simulink model "pmsm_mpc_simulink"  (R2022b)
settings: Solver=ode4  StartTime=0.0  StopTime=2  FixedStep=1e-05  RelTol=1e-3
values from neighbouring files (symbols this model uses):
  fault = evalin('base', 'fault')    [run_simulink_simulation.m]
  motor = evalin('base', 'motor')    [run_simulink_mpc_simulation.m]
  profile = evalin('base', 'profile')    [run_simulink_mpc_simulation.m]    (also in run_simulink_simulation.m)
settings Model: Creator=arpankailashgupta  LastModifiedBy=arpankailashgupta
settings DataIOCC: SaveOutput=off

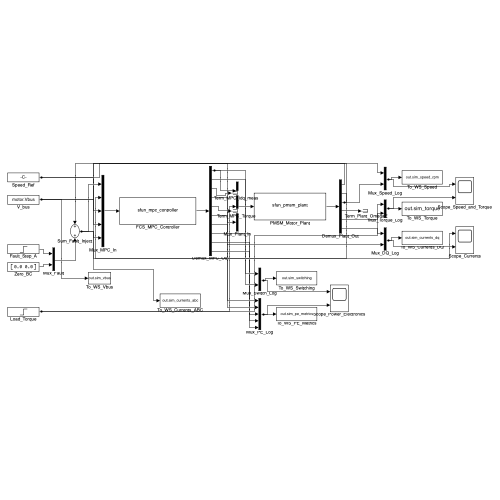
[thumbnail: Simulink's stored preview of the top-level diagram]
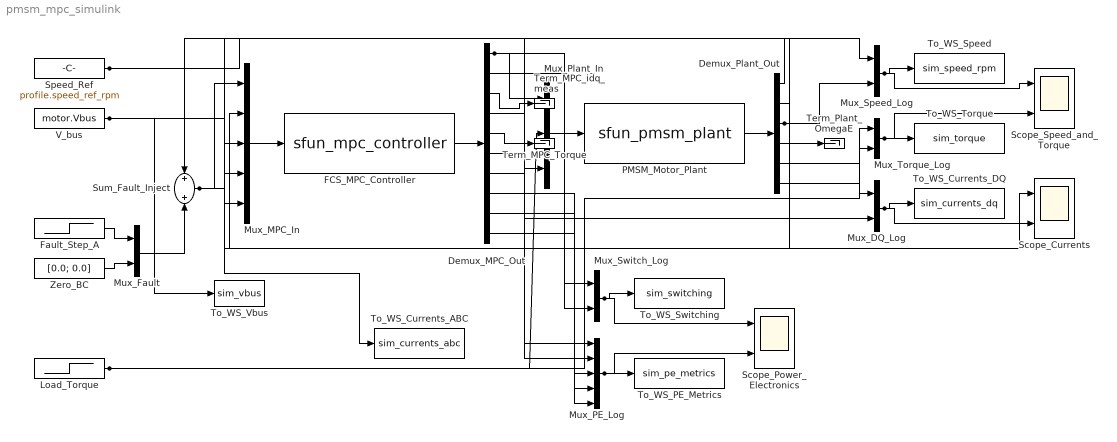
== system pmsm_mpc_simulink ==
  Demux_MPC_Out : Demux  Outputs=[3, 1, 2, 2, 1, 1, 1, 1, 1, 1]
  Demux_Plant_Out : Demux  Outputs=[3, 1, 1, 1, 1, 2]
  FCS_MPC_Controller : S-Function  FunctionName=sfun_mpc_controller  Parameters=sim_cfg.Ts_ctrl  SFunctionDeploymentMode=off  EnableBusSupport=off
  Fault_Step_A : Step  Time=fault.onset_time  Before=0.0  After=fault.offset_val * fault.enable  SampleTime=0
  Load_Torque : Step  Time=profile.load_step_time  Before=0.0  After=profile.load_torque_Nm  SampleTime=0
  Mux_DQ_Log : Mux  Inputs=2
  Mux_Fault : Mux  Inputs=2
  Mux_MPC_In : Mux  Inputs=5
  Mux_PE_Log : Mux  Inputs=5
  Mux_Plant_In : Mux  Inputs=3
  Mux_Speed_Log : Mux  Inputs=2
  Mux_Switch_Log : Mux  Inputs=2
  Mux_Torque_Log : Mux  Inputs=2
  PMSM_Motor_Plant : S-Function  FunctionName=sfun_pmsm_plant  Parameters=MotorParamVec, motor.Tcog  SFunctionDeploymentMode=off  EnableBusSupport=off
  Scope_Currents : Scope  NumInputPorts=2
  Scope_Power_Electronics : Scope  NumInputPorts=2
  Scope_Speed_and_Torque : Scope  NumInputPorts=2
  Speed_Ref : Constant  Value=profile.speed_ref_rpm
  Sum_Fault_Inject : Sum
  Term_MPC_Torque : Terminator
  Term_MPC_idq_meas : Terminator
  Term_Plant_OmegaE : Terminator
  To_WS_Currents_ABC : ToWorkspace  VariableName=sim_currents_abc  SampleTime=-1
  To_WS_Currents_DQ : ToWorkspace  VariableName=sim_currents_dq  SampleTime=-1
  To_WS_PE_Metrics : ToWorkspace  VariableName=sim_pe_metrics  SampleTime=-1
  To_WS_Speed : ToWorkspace  VariableName=sim_speed_rpm  SampleTime=-1
  To_WS_Switching : ToWorkspace  VariableName=sim_switching  SampleTime=-1
  To_WS_Torque : ToWorkspace  VariableName=sim_torque  SampleTime=-1
  To_WS_Vbus : ToWorkspace  VariableName=sim_vbus  SampleTime=-1
  V_bus : Constant  Value=motor.Vbus
  Zero_BC : Constant  Value=[0.0; 0.0]
  wires:
  Fault_Step_A/1 -> Mux_Fault/1
  Zero_BC/1 -> Mux_Fault/2
  Demux_Plant_Out/1 -> Sum_Fault_Inject/1
  Mux_Fault/1 -> Sum_Fault_Inject/2
  Sum_Fault_Inject/1 -> Mux_MPC_In/1, To_WS_Currents_ABC/1, Scope_Currents/1
  Demux_Plant_Out/2 -> Mux_MPC_In/2
  Demux_Plant_Out/3 -> Mux_MPC_In/3, Mux_Speed_Log/2
  Speed_Ref/1 -> Mux_MPC_In/4, Mux_Speed_Log/1
  V_bus/1 -> Mux_MPC_In/5, Mux_Plant_In/3, To_WS_Vbus/1
  Mux_MPC_In/1 -> FCS_MPC_Controller/1
  FCS_MPC_Controller/1 -> Demux_MPC_Out/1
  Demux_MPC_Out/1 -> Mux_Plant_In/1, Mux_Switch_Log/1
  Load_Torque/1 -> Mux_Plant_In/2, Mux_Torque_Log/2
  Mux_Plant_In/1 -> PMSM_Motor_Plant/1
  PMSM_Motor_Plant/1 -> Demux_Plant_Out/1
  Mux_Speed_Log/1 -> To_WS_Speed/1, Scope_Speed_and_Torque/1
  Demux_Plant_Out/5 -> Mux_Torque_Log/1
  Mux_Torque_Log/1 -> To_WS_Torque/1, Scope_Speed_and_Torque/2
  Demux_Plant_Out/6 -> Mux_DQ_Log/1
  Demux_MPC_Out/4 -> Mux_DQ_Log/2
  Mux_DQ_Log/1 -> To_WS_Currents_DQ/1, Scope_Currents/2
  Demux_MPC_Out/2 -> Mux_Switch_Log/2
  Mux_Switch_Log/1 -> To_WS_Switching/1, Scope_Power_Electronics/1
  Demux_MPC_Out/6 -> Mux_PE_Log/1
  Demux_MPC_Out/7 -> Mux_PE_Log/2
  Demux_MPC_Out/8 -> Mux_PE_Log/3
  Demux_MPC_Out/9 -> Mux_PE_Log/4
  Demux_MPC_Out/10 -> Mux_PE_Log/5
  Mux_PE_Log/1 -> To_WS_PE_Metrics/1, Scope_Power_Electronics/2
  Demux_Plant_Out/4 -> Term_Plant_OmegaE/1
  Demux_MPC_Out/3 -> Term_MPC_idq_meas/1
  Demux_MPC_Out/5 -> Term_MPC_Torque/1
